simulink library "Suspension_Utilities"  (R2025a)
settings: Solver=VariableStepAuto  StartTime=0.0  StopTime=10.0  RelTol=1e-3
undefined symbols (not defined in the file or in its folder): Ac, Af, Ar, hp1, hp2, hp3, hp_in, hp_in_f_ua, hp_in_r_ua, hp_mount_subframe, hp_shk_frame, hp_spr_bot, hp_spr_top, hpb, hpf, hpo, hpx, hpz, Newton, Raphson, rotYAxis, SubframeConnection, Upper_Arm_to_Subframe, Visual, X, Y, Z
libraries: sm_lib x75, $bdroot x23, linkage_bushing_6DOF_lib x13, fl_lib x4, sharedtransformsys x3, linkage_bushing_5DOF_lib x2, nesl_utility x1
(part 1 of 3)
Description:
  | Simscape Vehicle Templates Library
  | 
  | Copyright 2018-2026 The MathWorks, Inc.
settings Model: Creator=smiller  LastModifiedBy=smiller
settings OptimizationCC: ReuseModelBlockBuffer=off
settings ModelReferenceCC: EnableRefExpFcnMdlSchedulingChecks=on
settings RTWCC: GPUComputeCapability=3.5

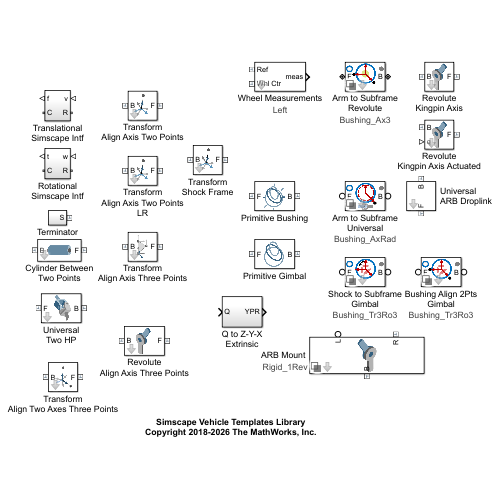
[thumbnail: Simulink's stored preview of the top-level diagram]
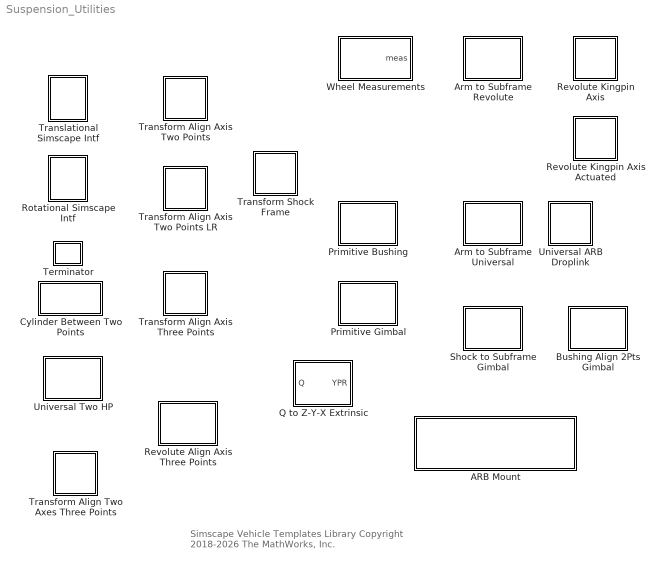
== system Suspension_Utilities ==
  note: Simscape Vehicle Templates Library
      | Copyright 2018-2026 The MathWorks, Inc.
  ARB Mount : Subsystem  Variant=on  VariantControlMode=label  VariantControl=Choice  LabelModeActiveChoice=Rigid_1Rev  mask{Connection=SubframeConnection, VariantLabel=SubframeConnection.class.Value}
      mask prompts: Connection "Connection Parameters"; VariantLabel "Variant Label"
      mask init:
      | curblk = gcb;
      | 
      | % Set variant for this block 
      | set_param(curblk,'LabelModeActiveChoice',VariantLabel);
      settings: AttributesFormatString=%<LabelModeActiveChoice>
  Arm to Subframe Revolute : Subsystem  Variant=on  VariantControlMode=label  VariantControl=Variant1  LabelModeActiveChoice=Bushing_Ax3  mask{popup_leftRight=Left, hp_f=hp_in_f_ua, hp_r=hp_in_r_ua, Connection=Upper_Arm_to_Subframe, VariantLabel=Upper_Arm_to_Subframe.class.Value}
      mask prompts: popup_leftRight "Left/Right"; hp_f "HP Front [x y z] (m)"; hp_r "HP Rear [x y z] (m)"; Connection "Connection Parameters"; VariantLabel "Variant Label"
      mask init:
      | curblk = gcb;
      | 
      | % Set variant for this block 
      | set_param(curblk,'LabelModeActiveChoice',VariantLabel);
      | 
      | if(popup_leftRight == 1)
      |     rhs_y = 1;
      | elseif(popup_leftRight == 2)
      |     rhs_y = -1;
      | end
      | 
      | rhs_hp = [1 rhs_y 1];
      settings: AttributesFormatString=%<ActiveVariant>
      mask TypeOptions popup_leftRight: Left | Right
      mask Display:
      | curblk = gcb;
      | activeVar = get_param(curblk,'activevariant');
      | ActiveVarCmd = get_param([curblk '/' strrep(activeVar,'_',' ')],'MaskDisplay');
      | eval(ActiveVarCmd);
  Arm to Subframe Universal : Subsystem  Variant=on  VariantControlMode=label  VariantControl=Variant1  LabelModeActiveChoice=Bushing_AxRad  mask(Universal Joint (Kinematic) or Compliant Element){popup_leftRight=Left, hp_joint=hp_in_f_ua, Connection=Upper_Arm_to_Subframe, VariantLabel=Upper_Arm_to_Subframe.class.Value, checkbox_setTargets=off}
      mask prompts: popup_leftRight "Left/Right"; hp_joint "Joint HP [x  y z] (m)"; Connection "Connection Parameters"; VariantLabel "Variant Label"; checkbox_setTargets "Set position targets to 0"
      mask help: Configurable part connection permitting two rotational degrees of freedom (Universal Joint) or a compliant connection. If "Right" is selected, y components will have their sign flipped.
      mask init:
      | curblk = gcb;
      | 
      | % Set variant for this block 
      | set_param(curblk,'LabelModeActiveChoice',VariantLabel);
      | 
      | set_param([curblk '/' strrep(VariantLabel,'_',' ')],'checkbox_setTargets',checkbox_setTargets);
      | 
      | if(popup_leftRight == 1)
      |     rhs_y = 1;
      | elseif(popup_leftRight == 2)
      |     rhs_y = -1;
      | end
      | 
      | rhs_hp = [1 rhs_y 1];
      settings: AttributesFormatString=%<ActiveVariant>
      mask TypeOptions popup_leftRight: Left | Right
  Bushing Align 2Pts Gimbal : Subsystem  Variant=on  VariantControlMode=label  VariantControl=Variant1  LabelModeActiveChoice=Bushing_Tr3Ro3  mask(Gimbal Joint (Kinematic) or Compliant Element){popup_leftRight=Left, hp_joint=0, Connection=Upper_Arm_to_Subframe, VariantLabel=Upper_Arm_to_Subframe.class.Value, checkbox_setTargets=off}
      mask prompts: popup_leftRight "Left/Right"; hp_joint "Joint HP [xyz] (m)"; Connection "Connection Parameters"; VariantLabel "Variant Label"; checkbox_setTargets "Set bushing joint targets to 0"
      mask help: Configurable part connection permitting three rotational degrees of freedom (Gimbal Joint) or a compliant connection. If "Right" is selected, y components will have their sign flipped.
      mask init:
      | curblk = gcb;
      | 
      | % Set variant for this block 
      | set_param(curblk,'LabelModeActiveChoice',VariantLabel);
      | 
      | if(popup_leftRight == 1)
      |     rhs_y = 1;
      | elseif(popup_leftRight == 2)
      |     rhs_y = -1;
      | end
      | 
      | rhs_hp = [1 rhs_y 1];
      | 
      | set_param([curblk '/Bushing Tr3Ro3'],'checkbox_setTargets',checkbox_setTargets);
      settings: AttributesFormatString=%<ActiveVariant>
      mask TypeOptions popup_leftRight: Left | Right
      mask Display:
      | curblk = gcb;
      | activeVar = get_param(curblk,'activevariant');
      | ActiveVarCmd = get_param([curblk '/' strrep(activeVar,'_',' ')],'MaskDisplay');
      | eval(ActiveVarCmd);
  Cylinder Between Two Points : Subsystem  mask(Cylinder between two points){hp_b=hpb, hp_f=hpf, Mass=1, clr_solid=[0.2 0.4 0.6], opc_solid=0.5, rad_solid=0.1}
      mask prompts: hp_b "Hardpoint at B [xyz] (m)"; hp_f "Hardpoint at F [xyz] (m)"; Mass "Mass (kg)"; clr_solid "Color [RGB]"; opc_solid "Opacity (0-1)"; rad_solid "Radius (m)"
      mask help: Models a cylinder parameterized by its end points.
      mask init:
      | [xftheta, xfaxis] = alignZAxisToLine(hp_b, hp_f);
      mask TypeOptions Mass: Solid/Mass
      mask TypeOptions clr_solid: Solid/GraphicDiffuseColor
      mask TypeOptions opc_solid: Solid/GraphicOpacity
      mask TypeOptions rad_solid: Solid/CylinderRadius
      mask DialogControl cont_vis Prompt: Visualization
      mask Display: image('sm_car_cylinder_two_points.png')
  Primitive Bushing : Subsystem
      mask Display: image('sm_car_primitive_bushing.png');
  Primitive Gimbal : Subsystem
      mask Display: image('sm_car_primitive_gimbal.png')
  Q to Z-Y-X Extrinsic : Subsystem
  Revolute Align Axis Three Points : Subsystem  mask(Revolute Joint 3 Points){popup_leftRight=Left, hp_1=[0 0 0], hp_2=[1 0 1], hp_3=[0 1 1], positionTargetSpecify=off, PositionTargetValue=0}
      mask prompts: popup_leftRight "Left/Right"; hp_1 "Hardpoint 1 [xyz] (m)"; hp_2 "Hardpoint 2 [xyz] (m)"; hp_3 "Hardpoint 3 [xyz] (m)"; positionTargetSpecify "Position Target Specify"; PositionTargetValue "Joint Target Value (deg)"
      mask help:
      | Revolute Joint with degree of freedom normal to 3 hardpoints.
      |
      | Positive z-axis will point along cross (HP1 -> HP3, HP1->HP2).
      mask init:
      | % Set parameter for mirroring (+y or -y)
      | if(popup_leftRight == 1)
      |     rhs_susp = 1;
      | elseif(popup_leftRight == 2)
      |     rhs_susp = -1;
      | end
      | rhs_hp = [1 rhs_susp 1];
      | 
      | if(popup_leftRight == 1)
      |     set_param([gcb '/Transform Align Axis B'],'popup_f_axis','+Z');
      |     set_param([gcb '/Transform Align Axis F'],'popup_f_axis','+Z');
      | elseif(popup_leftRight == 2)
      |     set_param([gcb '/Transform Align Axis B'],'popup_f_axis','-Z');
      |     set_param([gcb '/Transform Align Axis F'],'popup_f_axis','-Z');
      | end
      | 
      | if(get_param(gcb,'positionTargetSpecify'))
      |     set_param([gcb '/Revolute Bellcrank Pivot'],'PositionTargetSpecify','on')
      | else
      |     set_param([gcb '/Revolute Joint'],'PositionTargetSpecify','off')
      | end
      mask TypeOptions popup_leftRight: Left | Right
      mask TypeOptions PositionTargetValue:
      | Revolute
      | Bellcrank Pivot/PositionTargetValue
      mask Display: image('sm_car_variant_revolute.png')
  Revolute Kingpin Axis : Subsystem  mask{popup_leftRight=Left, aCaster=0, aKPI=0}
      mask prompts: popup_leftRight "Left/Right"; aCaster "Caster Angle (deg)"; aKPI "King Pin Inclination (KPI) Angle (deg)"
      mask init:
      | if(popup_leftRight == 1)
      |     rhs_KPIsign = 1;
      | elseif(popup_leftRight == 2)
      |     rhs_KPIsign = -1;
      | end
      mask TypeOptions popup_leftRight: Left | Right
      mask DialogControl text_caster Prompt: Positive Caster: Top Rear of WC
      mask DialogControl text_kpi Prompt: Positive KPI: Top Inside Bottom
      mask Display: image('sm_car_rev_joint_IMAGE.png');
  Revolute Kingpin Axis Actuated : Subsystem  mask{popup_leftRight=Left, aCaster=0, aKPI=0}
      mask prompts: popup_leftRight "Left/Right"; aCaster "Caster Angle (deg)"; aKPI "King Pin Inclination (KPI) Angle (deg)"
      mask init:
      | if(popup_leftRight == 1)
      |     rhs_KPIsign = 1;
      | elseif(popup_leftRight == 2)
      |     rhs_KPIsign = -1;
      | end
      mask TypeOptions popup_leftRight: Left | Right
      mask DialogControl text_caster Prompt: Positive Caster: Top Rear of WC
      mask DialogControl text_kpi Prompt: Positive KPI: Top Inside Bottom
      mask Display: image('sm_car_rev_joint_IMAGE.png');
  Rotational Simscape Intf : Subsystem
  Shock to Subframe Gimbal : Subsystem  Variant=on  VariantControlMode=label  VariantControl=Variant1  LabelModeActiveChoice=Bushing_Tr3Ro3  mask{popup_leftRight=Left, Connection=Upper_Arm_to_Subframe, VariantLabel=Upper_Arm_to_Subframe.class.Value, checkbox_setTargets=on}
      mask prompts: popup_leftRight "Left/Right"; Connection "Connection Parameters"; VariantLabel "Variant Label"; checkbox_setTargets "Set bushing joint targets to 0"
      mask init:
      | curblk = gcb;
      | 
      | % Set variant for this block 
      | set_param(curblk,'LabelModeActiveChoice',VariantLabel);
      | 
      | if(popup_leftRight == 1)
      |     rhs_y = 1;
      | elseif(popup_leftRight == 2)
      |     rhs_y = -1;
      | end
      | 
      | set_param([curblk '/Bushing Tr3Ro3'],'checkbox_setTargets',checkbox_setTargets);
      settings: AttributesFormatString=%<ActiveVariant>
      mask TypeOptions popup_leftRight: Left | Right
      mask Display:
      | curblk = gcb;
      | activeVar = get_param(curblk,'activevariant');
      | ActiveVarCmd = get_param([curblk '/' strrep(activeVar,'_',' ')],'MaskDisplay');
      | eval(ActiveVarCmd);
  Terminator : Subsystem
  Transform Align Axis Three Points : Subsystem  mask(Transform Align Axis Three Points){pt1=hp1, pt2=hp2, pt3=hp3, popup_f_axis=+Z}
      mask prompts: pt1 "Point 1 [xyz] (m)"; pt2 "Point 2 [xyz] (m)"; pt3 "Point 3 [xyz] (m)"; popup_f_axis "Axis of F Frame to Aim at Target"
      mask help: Transforms a frame to aim a selected axis along a normal to a plane defined by 3 points. All points must be defined relative to the same reference frame. Normal to the plane is defined as cross (HP1 -> HP3, HP1->HP2).
      mask init:
      | switch popup_f_axis
      |     case 1, vec = [ 1  0  0];
      |     case 2, vec = [ 0  1  0];
      |     case 3, vec = [ 0  0  1];
      |     case 4, vec = [-1  0  0];
      |     case 5, vec = [ 0 -1  0];
      |     case 6, vec = [ 0  0 -1];
      | end
      | 
      | % Unit vectors 
      | uvec1 = (pt3-pt1)/norm(pt3-pt1);
      | uvec2 = (pt2-pt1)/norm(pt2-pt1);
      | 
      | nvec = cross(uvec1,uvec2);
      | unvec = nvec/norm(nvec);
      | 
      | % Force nvec to point along +z
      | %if(unvec(3)<0)
      | %    unvec = -unvec;
      | %end
      | rotaxis = cross(vec,unvec);
      | 
      | if (norm(rotaxis)==0)
      |     if (sum(uvec1==0)==3 || sum(uvec2==0)==3)  % hps collocated
      |         rotangle = 0; 
      |     elseif ((sum(uvec1+uvec2)==0) ...  % vectors antiparallel    
      |             || (sum(vec+unvec))==0)    % vec and unvec antiparallel
      |         rotangle = pi;
      |         rotaxis = circshift(vec,1);
      |     else                       % vectors parallel
      |         rotangle = 0;          
      |     end
      | else
      |     rotangle = acos(dot(vec,unvec));
      |     %rotangle = acos(dot(vec,(hp_t-hp_b)/norm((hp_t-hp_b))))
      | end
      mask TypeOptions popup_f_axis: +X | +Y | +Z | -X | -Y | -Z
      mask Display: image('sm_car_transform_align_axis_three_points.png')
  Transform Align Axis Two Points : Subsystem  mask(Transform Align Axis Two Points){hp_b=hp1, hp_t=hp2, popup_f_axis=-Z}
      mask prompts: hp_b "Location of B [xyz] (m)"; hp_t "Target for Frame Axis [xyz] (m)"; popup_f_axis "Axis of F Frame to Aim at Target"
      mask help: Transforms a frame to aim a selected axis at a target point. Both points must be defined relative to the same reference frame.
      mask init:
      | switch popup_f_axis
      |     case 1, vec = [ 1  0  0];
      |     case 2, vec = [ 0  1  0];
      |     case 3, vec = [ 0  0  1];
      |     case 4, vec = [-1  0  0];
      |     case 5, vec = [ 0 -1  0];
      |     case 6, vec = [ 0  0 -1];
      | end
      | 
      | uvec_bt = (hp_t-hp_b)/norm(hp_t-hp_b);
      | rotaxis = cross(vec,uvec_bt);
      | 
      | if (norm(rotaxis)==0)
      |     if (uvec_bt==0)            % hps collocated
      |         rotangle = 0; 
      |     elseif ((uvec_bt+vec)==0)  % vectors antiparallel    
      |         rotangle = pi;
      |         rotaxis = circshift(vec,1);
      |     else                       % vectors parallel
      |         rotangle = 0;          
      |     end
      | else
      |     rotangle = acos(dot(vec,uvec_bt));
      |     %rotangle = acos(dot(vec,(hp_t-hp_b)/norm((hp_t-hp_b))))
      | end
      mask TypeOptions popup_f_axis: +X | +Y | +Z | -X | -Y | -Z
      mask Display: image('sm_car_transform_align_axis_two_points.png')
  Transform Align Axis Two Points LR : Subsystem  mask{popup_leftRight=Left, hp_spr_top=hp_spr_top, hp_spr_bot=hp_spr_bot}
      mask prompts: popup_leftRight "Left/Right"; hp_spr_top "Spring Top [xyz] (m)"; hp_spr_bot "Spring Bottom [xyz] (m)"
      mask init:
      | if(popup_leftRight == 1)
      |     rhs_y = 1;
      | elseif(popup_leftRight == 2)
      |     rhs_y = -1;
      | end
      | 
      | rhs_hp = [1 rhs_y 1];
      mask TypeOptions popup_leftRight: Left | Right
      mask Display: image('sm_car_transform_align_axis_two_points.png')
  Transform Align Two Axes Three Points : Subsystem  mask(Transform Align Two Axes Three Points){hpo=hpo, hpz=hpz, hpx=hpx}
      mask prompts: hpo "Origin [x y z] (m)"; hpz "Point to align z-axis [x y z] (m)"; hpx "Point to align x-axis [x y z] (m)"
      mask help: Transforms a frame to aim two selected axes to point at two provided points. All points must be defined relative to the same reference frame.
      mask init:
      | R = frameRotationFromTwoPoints(hpo, hpz, hpx);
      mask Display: image('sm_car_transform_align_two_axes_three_points.png')
  Transform Shock Frame : Subsystem  mask{popup_leftRight=Left, hp_spr_top=hp_spr_top, hp_spr_bot=hp_spr_bot, hp_shk_frame=hp_shk_frame}
      mask prompts: popup_leftRight "Left/Right"; hp_spr_top "Shock Top [xyz] (m)"; hp_spr_bot "Shock Bottom [xyz] (m)"; hp_shk_frame "Shock Frame [xyz] (m)"
      mask init:
      | if(popup_leftRight == 1)
      |     rhs_y = 1;
      | elseif(popup_leftRight == 2)
      |     rhs_y = -1;
      | end
      | 
      | vecBotTop = hp_spr_top-hp_spr_bot;
      | 
      | qx = atan2(vecBotTop(2),vecBotTop(3));
      | qy = atan2(vecBotTop(1),vecBotTop(3));
      | 
      | R = frameRotationXYextr(qx*rhs_y,qy);
      mask TypeOptions popup_leftRight: Left | Right
      mask Display: image('sm_car_transform_align_axis_two_points.png')
  Translational Simscape Intf : Subsystem
  Universal ARB Droplink : Subsystem  mask{rotYAxis=rotYAxis}
      mask prompts: rotYAxis "Universal Y Rotation (deg)"
  Universal Two HP : Subsystem  mask{popup_leftRight=Left, hp_f=hp_in_f_ua, hp_r=hp_in_r_ua}
      mask prompts: popup_leftRight "Left/Right"; hp_f "HP Front [xyz] (m)"; hp_r "HP Rear [xyz] (m)"
      mask init:
      | if(popup_leftRight == 1)
      |     rhs_y = 1;
      | elseif(popup_leftRight == 2)
      |     rhs_y = -1;
      | end
      | 
      | rhs_hp = [1 rhs_y 1];
      mask TypeOptions popup_leftRight: Left | Right
      mask Display: image('sm_car_variant_universal.png');
  Wheel Measurements : Subsystem  mask(Wheel Measurements){popup_leftRight=Left}
      mask prompts: popup_leftRight "Left/Right"
      mask help: Calculates toe and camber angles based on orientation of wheel spin axis. To estimate steering axis inclination, the same measurements are done along the longitudinal axis (X) of the tire. Set Left/Right so that the sign of the logged toe and camber angles is associated with towards/away from vehicle center.
      mask init:
      | if(popup_leftRight == 1)
      |     rhs_tc = 1;
      | elseif(popup_leftRight == 2)
      |     rhs_tc = -1;
      | end
      settings: AttributesFormatString=%<popup_leftRight>
      mask TypeOptions popup_leftRight: Left | Right

== system Suspension_Utilities/ARB Mount ==
  Bushing Ax3 : Subsystem  VariantControl=Bushing_Ax3  mask{hp_j=hp_mount_subframe, Bushing=Connection}
      mask prompts: hp_j "Joint HP [x  y z] (m)"; Bushing "Parameters (struct)"
      mask init:
      | %{
      | set_param([gcb '/Bushing L'],...
      |     'popup_force_law_spr_axiX', sprx.Law.Value,...
      |     'popup_force_law_spr_axiY', spry.Law.Value,...
      |     'popup_force_law_spr_axiZ', sprz.Law.Value,...
      |     'popup_force_law_dam_axiX', damx.Law.Value,...
      |     'popup_force_law_dam_axiY', damy.Law.Value,...
      |     'popup_force_law_dam_axiZ', damz.Law.Value...
      |     );
      | 
      | set_param([gcb '/Bushing R'],...
      |     'popup_force_law_spr_axiX', sprx.Law.Value,...
      |     'popup_force_law_spr_axiY', spry.Law.Value,...
      |     'popup_force_law_spr_axiZ', sprz.Law.Value,...
      |     'popup_force_law_dam_axiX', damx.Law.Value,...
      |     'popup_force_law_dam_axiY', damy.Law.Value,...
      |     'popup_force_law_dam_axiZ', damz.Law.Value...
      |     );
      | %}
      mask Display: image('sm_car_subframe_arb_bushing_2tra_perpaxial.png');
  Bushing Tr3Ro3 : Subsystem  VariantControl=Bushing_Tr3Ro3  mask{Bushing=Connection, sprx_law=Connection.SpringX.Law.Value, spry_law=Connection.SpringY.Law.Value, sprz_law=Connection.SpringZ.Law.Value, damx_law=Connection.DamperX.Law.Value, damy_law=Connection.DamperY.Law.Value, damz_law=Connection.DamperZ.Law.Value, sprx_law_rot=Connection.SpringX.Law.Value, spry_law_rot=Connection.SpringY.Law.Value, sprz_law_rot=Connection.SpringZ.Law.Value, damx_law_rot=Connection.DamperX.Law.Value, damy_law_rot=Connection.DamperY.Law.Value, damz_law_rot=Connection.DamperZ.Law.Value}
      mask prompts: Bushing "Parameters (struct)"; sprx_law "Spring X Force Law"; spry_law "Spring Y Force Law"; sprz_law "Spring Z Force Law"; damx_law "Damper X Force Law"; damy_law "Damper Y Force Law"; damz_law "Damper Z Force Law"; sprx_law_rot "Spring X Force Law"; spry_law_rot "Spring Y Force Law"; sprz_law_rot "Spring Z Force Law"; damx_law_rot "Damper X Force Law"; damy_law_rot "Damper Y Force Law"; damz_law_rot "Damper Z Force Law"
      mask init:
      | %{
      | set_param([gcb '/Bushing L'],...
      |     'popup_force_law_spr_axiX', sprx_law,...
      |     'popup_force_law_spr_axiY', spry_law,...
      |     'popup_force_law_spr_axiZ', sprz_law,...
      |     'popup_force_law_dam_axiX', damx_law,...
      |     'popup_force_law_dam_axiY', damy_law,...
      |     'popup_force_law_dam_axiZ', damz_law,...
      |     'popup_force_law_spr_torX', sprx_law_rot,...
      |     'popup_force_law_spr_torY', spry_law_rot,...
      |     'popup_force_law_spr_torZ', sprz_law_rot,...
      |     'popup_force_law_dam_torX', damx_law_rot,...
      |     'popup_force_law_dam_torY', damy_law_rot,...
      |     'popup_force_law_dam_torZ', damz_law_rot...
      |     );
      | 
      | set_param([gcb '/Bushing R'],...
      |     'popup_force_law_spr_axiX', sprx_law,...
      |     'popup_force_law_spr_axiY', spry_law,...
      |     'popup_force_law_spr_axiZ', sprz_law,...
      |     'popup_force_law_dam_axiX', damx_law,...
      |     'popup_force_law_dam_axiY', damy_law,...
      |     'popup_force_law_dam_axiZ', damz_law,...
      |     'popup_force_law_spr_torX', sprx_law_rot,...
      |     'popup_force_law_spr_torY', spry_law_rot,...
      |     'popup_force_law_spr_torZ', sprz_law_rot,...
      |     'popup_force_law_dam_torX', damx_law_rot,...
      |     'popup_force_law_dam_torY', damy_law_rot,...
      |     'popup_force_law_dam_torZ', damz_law_rot...
      |     );
      | %}
      mask DialogControl cont_trans Prompt: Translational
      mask DialogControl cont_rot Prompt: Rotational
      mask Display: image('sm_car_subframe_arb_bushing_2tra3rot_qz.png');
  Rigid 1Rev : Subsystem  VariantControl=Rigid_1Rev
      mask Display: image('sm_car_subframe_arb_rev.png');
  L : PMIOPort  Side=Right
  R : PMIOPort  Port=2  Side=Right
  B : PMIOPort  Port=3  Side=Left

== system Suspension_Utilities/Arm to Subframe Revolute ==
  Bushing Ax3 : Subsystem  VariantControl=Bushing_Ax3  mask{Bushing=Connection}
      mask prompts: Bushing "Parameters (struct)"
      mask Display: image('sm_car_bushing_tr3_perpaxial.png');
  Bushing AxRad : Subsystem  VariantControl=Bushing_AxRad  mask{Bushing=Connection}
      mask prompts: Bushing "Parameters (struct)"
      mask Display: image('sm_car_bushing_axrad_6dof.png');
  Bushing Tr3Ro3 : Subsystem  VariantControl=Bushing_Tr3Ro3  mask{Bushing=Connection}
      mask prompts: Bushing "Parameters (struct)"
      mask Display: image('sm_car_bushing_tr3ro3_2pts.png');
  Rigid 1Rev : Subsystem  VariantControl=Rigid_1Rev
      mask Display: image('sm_car_variant_revolute.png')
  Rigid 2Rev : Subsystem  VariantControl=Rigid_2Rev
      mask Display: image('sm_car_variant_revolute_2rev.png');
  F : PMIOPort  Side=Right
  " B" : PMIOPort  Port=2  Side=Left

== system Suspension_Utilities/Arm to Subframe Universal ==
  Bushing Ax3 : linkage_bushing_5DOF_lib/Bushing Ax3  VariantControl=Bushing_Ax3  leftOrRight=rhs_y  hp_j=hp_joint  checkbox_setTargets=on  hp_z=Connection.sAxialOrientationZ.Value  hp_x=Connection.sAxialOrientationX.Value  AxisAttachment=Connection.AxisAttachment.class.Value  sprx=Connection.SpringX  spry=Connection.SpringY  sprz=Connection.SpringZ  damx=Connection.DamperX  damy=Connection.DamperY  damz=Connection.DamperZ  shell_or=Visual.hp.rad*2  shell_ir=Visual.hp.rad  shell_len=Visual.hp.rad*2  elastomer_clr=Visual.Bushing.clr  elastomer_opc=Visual.part.opc  shell_clr=Visual.BushingShell.clr  shell_opc=Visual.part.opc  sleeve_clr=Visual.Bushing.clr  sleeve_opc=Visual.part.opc
  Bushing AxRad : linkage_bushing_5DOF_lib/Bushing AxRad  VariantControl=Bushing_AxRad  leftOrRight=rhs_y  hp_j=hp_joint  checkbox_setTargets=on  hp_z=Connection.sAxialOrientation.Value  sprRad=Connection.RadialSpring  damRad=Connection.RadialDamper  sprAxi=Connection.AxialSpring  damAxi=Connection.AxialDamper  shell_or=Visual.hp.rad*2  shell_len=Visual.hp.rad*2  shell_clr=Visual.BushingShell.clr  shell_opc=Visual.part.opc  sleeve_clr=Visual.Bushing.clr  sleeve_opc=Visual.part.opc
  Bushing Tr3Ro3 : linkage_bushing_6DOF_lib/Bushing Tr3Ro3 2Pts  VariantControl=Bushing_Tr3Ro3  checkbox_setTargets=off  leftOrRight=rhs_y  hp_j=hp_joint  hp_z=Connection.sAxialOrientationZ.Value  hp_x=Connection.sAxialOrientationX.Value  sprx=Connection.SpringX  spry=Connection.SpringY  sprz=Connection.SpringZ  damx=Connection.DamperX  damy=Connection.DamperY  damz=Connection.DamperZ  sprqx=Connection.SpringqX  sprqy=Connection.SpringqY  sprqz=Connection.SpringqZ  damqx=Connection.DamperqX  damqy=Connection.DamperqY  damqz=Connection.DamperqZ  shell_or=Visual.hp.rad*2  shell_len=Visual.hp.rad*2  shell_clr=Visual.BushingShell.clr  shell_opc=Visual.part.opc  sleeve_clr=Visual.Bushing.clr  sleeve_opc=Visual.part.opc
  Rigid UJ : Subsystem  VariantControl=Rigid_UJ  mask{popup_leftRight=Left, checkbox_setTargets=on}
      mask prompts: popup_leftRight "Left/Right"; checkbox_setTargets "Set position targets to 0"
      mask init:
      | curblk = gcb;
      | 
      | if(popup_leftRight == 1)
      |     rhs_y = 1;
      | elseif(popup_leftRight == 2)
      |     rhs_y = -1;
      | end
      | 
      | rhs_hp = [1 rhs_y 1];
      | 
      | if(checkbox_setTargets)
      |     set_param([curblk '/Universal Joint'],...
      |         'RxPositionTargetSpecify','on',...
      |         'RyPositionTargetSpecify','on'...
      |         );
      | else
      |     set_param([curblk '/Universal Joint'],...
      |         'RxPositionTargetSpecify','off',...
      |         'RyPositionTargetSpecify','off'...
      |         );
      | end
      mask TypeOptions popup_leftRight: Left | Right
      mask Display: image('sm_car_variant_universal.png');
  F : PMIOPort  Side=Right
  " B" : PMIOPort  Port=2  Side=Left

== system Suspension_Utilities/Bushing Align 2Pts Gimbal ==
  Bushing Tr3Ro3 : linkage_bushing_6DOF_lib/Bushing Tr3Ro3 2Pts  VariantControl=Bushing_Tr3Ro3  checkbox_setTargets=on  leftOrRight=rhs_y  hp_j=hp_joint  hp_z=Connection.sAxialOrientationZ.Value  hp_x=Connection.sAxialOrientationX.Value  sprx=Connection.SpringX  spry=Connection.SpringY  sprz=Connection.SpringZ  damx=Connection.DamperX  damy=Connection.DamperY  damz=Connection.DamperZ  sprqx=Connection.SpringqX  sprqy=Connection.SpringqY  sprqz=Connection.SpringqZ  damqx=Connection.DamperqX  damqy=Connection.DamperqY  damqz=Connection.DamperqZ  shell_or=Visual.hp.rad*2  shell_len=Visual.hp.rad*2  shell_clr=Visual.BushingShell.clr  shell_opc=Visual.part.opc  sleeve_clr=Visual.Bushing.clr  sleeve_opc=Visual.part.opc
  Rigid Gimbal : Subsystem  VariantControl=Rigid_Gimbal
      mask Display: image('sm_car_variant_bushing_gimbal.png')
  F : PMIOPort  Side=Right
  " B" : PMIOPort  Port=2  Side=Left

== system Suspension_Utilities/Cylinder Between Two Points ==
  Solid : sm_lib/Body Elements/Cylindrical Solid  CylinderRadius=rad_solid  CylinderRadiusUnits=m  CylinderLength=norm(hp_f-hp_b)  CylinderLengthUnits=m  ExportEntireGeometry=off  InertiaType=CalculateFromGeometry  BasedOnType=Mass  Density=1000  DensityUnits=kg/m^3  Mass=Mass  MassUnits=kg  CenterOfMass=[0 0 0]  CenterOfMassUnits=m  MomentsOfInertia=[1 1 1]  MomentsOfInertiaUnits=kg*m^2  ProductsOfInertia=[0 0 0]  ProductsOfInertiaUnits=kg*m^2  GraphicType=FromGeometry  MarkerShape=Sphere  MarkerSize=10  GraphicVisPropType=SimpleVisualProperties  GraphicDiffuseColor=clr_solid  GraphicOpacity=opc_solid  GraphicSpecularColor=[0.5 0.5 0.5 1.0]  GraphicAmbientColor=[0.15 0.15 0.15 1.0]  GraphicEmissiveColor=[0.0 0.0 0.0 1.0]  GraphicShininess=75  DoExposeReferenceFrame=on  SerializedFrames=<Frames/>
  Transform Align Z B to F : sm_lib/Frames and Transforms/Rigid Transform  RotationMethod=ArbitraryAxis  FollAlignAxisA=+X  BaseAlignAxisA=+Y  FollAlignAxisB=+Y  BaseAlignAxisB=+Z  RotationStandardAxis=+Z  RotationAngle=xftheta  RotationAngleUnits=rad  RotationArbitraryAxis=xfaxis  RotationSequenceAxes=FollowerAxes  RotationSequence=XYX  RotationSequenceAngles=[0 0 0]  RotationSequenceAnglesUnits=deg  RotationMatrix=[1 0 0; 0 1 0; 0 0 1]  Quaternion=[1 0 0 0]  TranslationMethod=None  TranslationCartesianOffset=[0 0 0]  TranslationCartesianOffsetUnits=m  TranslationStandardAxis=+Z  TranslationStandardOffset=0  TranslationStandardOffsetUnits=m  TranslationROffset=0  TranslationROffsetUnits=m  TranslationThetaOffset=0  TranslationThetaOffsetUnits=deg  TranslationZOffset=0  TranslationZOffsetUnits=m
  Transform B to Ctr : sm_lib/Frames and Transforms/Rigid Transform  RotationMethod=None  FollAlignAxisA=+X  BaseAlignAxisA=+Y  FollAlignAxisB=+Y  BaseAlignAxisB=+Z  RotationStandardAxis=+Z  RotationAngle=0.0  RotationAngleUnits=deg  RotationArbitraryAxis=[0 0 1]  RotationSequenceAxes=FollowerAxes  RotationSequence=XYX  RotationSequenceAngles=[0 0 0]  RotationSequenceAnglesUnits=deg  RotationMatrix=[1 0 0; 0 1 0; 0 0 1]  Quaternion=[1 0 0 0]  TranslationMethod=Cartesian  TranslationCartesianOffset=0.5*(hp_f-hp_b)  TranslationCartesianOffsetUnits=m  TranslationStandardAxis=+Z  TranslationStandardOffset=0  TranslationStandardOffsetUnits=m  TranslationROffset=0  TranslationROffsetUnits=m  TranslationThetaOffset=0  TranslationThetaOffsetUnits=deg  TranslationZOffset=0  TranslationZOffsetUnits=m
  Transform Ctr to F : sm_lib/Frames and Transforms/Rigid Transform  RotationMethod=None  FollAlignAxisA=+X  BaseAlignAxisA=+Y  FollAlignAxisB=+Y  BaseAlignAxisB=+Z  RotationStandardAxis=+Z  RotationAngle=0.0  RotationAngleUnits=deg  RotationArbitraryAxis=[0 0 1]  RotationSequenceAxes=FollowerAxes  RotationSequence=XYX  RotationSequenceAngles=[0 0 0]  RotationSequenceAnglesUnits=deg  RotationMatrix=[1 0 0; 0 1 0; 0 0 1]  Quaternion=[1 0 0 0]  TranslationMethod=Cartesian  TranslationCartesianOffset=0.5*(hp_f-hp_b)  TranslationCartesianOffsetUnits=m  TranslationStandardAxis=+Z  TranslationStandardOffset=0  TranslationStandardOffsetUnits=m  TranslationROffset=0  TranslationROffsetUnits=m  TranslationThetaOffset=0  TranslationThetaOffsetUnits=deg  TranslationZOffset=0  TranslationZOffsetUnits=m
  F : PMIOPort  Side=Right
  B : PMIOPort  Port=2  Side=Left
  connections:
  Transform Ctr to F/RConn1 -- F/RConn1
  Transform Align Z B to F/RConn1 -- Solid/RConn1
  Transform Align Z B to F/LConn1 -- Transform Ctr to F/LConn1 -- Transform B to Ctr/RConn1
  Transform B to Ctr/LConn1 -- B/RConn1

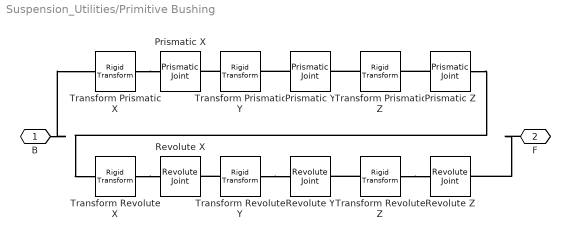
== system Suspension_Utilities/Primitive Bushing ==
  Prismatic X : sm_lib/Joints/Prismatic Joint  JointMode=Normal  CompositeWrenchDir=FollowerOnBase  CompositeWrenchFrame=BaseFrame  SenseConstraintForce=off  SenseConstraintTorque=off  SenseTotalForce=off  SenseTotalTorque=off  PositionTargetSpecify=off  PositionTargetPriority=High  PositionTargetValue=0  PositionTargetValueUnits=m  VelocityTargetSpecify=off  VelocityTargetPriority=High  VelocityTargetValue=0  VelocityTargetValueUnits=m/s  EquilibriumPosition=0  EquilibriumPositionUnits=m  SpringStiffness=0  SpringStiffnessUnits=N/m  DampingCoefficient=0  DampingCoefficientUnits=N/(m/s)  LowerLimitSpecify=off  LowerLimitBound=-1  LowerLimitBoundUnits=m  LowerLimitStiffness=1e6  LowerLimitStiffnessUnits=N/m  LowerLimitDamping=1e3  LowerLimitDampingUnits=N/(m/s)  LowerLimitTransitionRegionWidth=1e-4  LowerLimitTransitionRegionWidthUnits=m  UpperLimitSpecify=off  UpperLimitBound=1  UpperLimitBoundUnits=m  UpperLimitStiffness=1e6  UpperLimitStiffnessUnits=N/m  UpperLimitDamping=1e3  UpperLimitDampingUnits=N/(m/s)  UpperLimitTransitionRegionWidth=1e-4  UpperLimitTransitionRegionWidthUnits=m  TorqueActuationMode=NoTorque  MotionActuationMode=ComputedMotion  SensePosition=off  SenseVelocity=off  SenseAcceleration=off  SenseTorqueForce=off  SenseLowerLimitTorqueForce=off  SenseUpperLimitTorqueForce=off
  Prismatic Y : sm_lib/Joints/Prismatic Joint  JointMode=Normal  CompositeWrenchDir=FollowerOnBase  CompositeWrenchFrame=BaseFrame  SenseConstraintForce=off  SenseConstraintTorque=off  SenseTotalForce=off  SenseTotalTorque=off  PositionTargetSpecify=off  PositionTargetPriority=High  PositionTargetValue=0  PositionTargetValueUnits=m  VelocityTargetSpecify=off  VelocityTargetPriority=High  VelocityTargetValue=0  VelocityTargetValueUnits=m/s  EquilibriumPosition=0  EquilibriumPositionUnits=m  SpringStiffness=0  SpringStiffnessUnits=N/m  DampingCoefficient=0  DampingCoefficientUnits=N/(m/s)  LowerLimitSpecify=off  LowerLimitBound=-1  LowerLimitBoundUnits=m  LowerLimitStiffness=1e6  LowerLimitStiffnessUnits=N/m  LowerLimitDamping=1e3  LowerLimitDampingUnits=N/(m/s)  LowerLimitTransitionRegionWidth=1e-4  LowerLimitTransitionRegionWidthUnits=m  UpperLimitSpecify=off  UpperLimitBound=1  UpperLimitBoundUnits=m  UpperLimitStiffness=1e6  UpperLimitStiffnessUnits=N/m  UpperLimitDamping=1e3  UpperLimitDampingUnits=N/(m/s)  UpperLimitTransitionRegionWidth=1e-4  UpperLimitTransitionRegionWidthUnits=m  TorqueActuationMode=NoTorque  MotionActuationMode=ComputedMotion  SensePosition=off  SenseVelocity=off  SenseAcceleration=off  SenseTorqueForce=off  SenseLowerLimitTorqueForce=off  SenseUpperLimitTorqueForce=off
  Prismatic Z : sm_lib/Joints/Prismatic Joint  JointMode=Normal  CompositeWrenchDir=FollowerOnBase  CompositeWrenchFrame=BaseFrame  SenseConstraintForce=off  SenseConstraintTorque=off  SenseTotalForce=off  SenseTotalTorque=off  PositionTargetSpecify=off  PositionTargetPriority=High  PositionTargetValue=0  PositionTargetValueUnits=m  VelocityTargetSpecify=off  VelocityTargetPriority=High  VelocityTargetValue=0  VelocityTargetValueUnits=m/s  EquilibriumPosition=0  EquilibriumPositionUnits=m  SpringStiffness=0  SpringStiffnessUnits=N/m  DampingCoefficient=0  DampingCoefficientUnits=N/(m/s)  LowerLimitSpecify=off  LowerLimitBound=-1  LowerLimitBoundUnits=m  LowerLimitStiffness=1e6  LowerLimitStiffnessUnits=N/m  LowerLimitDamping=1e3  LowerLimitDampingUnits=N/(m/s)  LowerLimitTransitionRegionWidth=1e-4  LowerLimitTransitionRegionWidthUnits=m  UpperLimitSpecify=off  UpperLimitBound=1  UpperLimitBoundUnits=m  UpperLimitStiffness=1e6  UpperLimitStiffnessUnits=N/m  UpperLimitDamping=1e3  UpperLimitDampingUnits=N/(m/s)  UpperLimitTransitionRegionWidth=1e-4  UpperLimitTransitionRegionWidthUnits=m  TorqueActuationMode=NoTorque  MotionActuationMode=ComputedMotion  SensePosition=off  SenseVelocity=off  SenseAcceleration=off  SenseTorqueForce=off  SenseLowerLimitTorqueForce=off  SenseUpperLimitTorqueForce=off
  Revolute X : sm_lib/Joints/Revolute Joint  JointMode=Normal  CompositeWrenchDir=FollowerOnBase  CompositeWrenchFrame=BaseFrame  SenseConstraintForce=off  SenseConstraintTorque=off  SenseTotalForce=off  SenseTotalTorque=off  PositionTargetSpecify=off  PositionTargetPriority=High  PositionTargetValue=0  PositionTargetValueUnits=deg  VelocityTargetSpecify=off  VelocityTargetPriority=High  VelocityTargetValue=0  VelocityTargetValueUnits=deg/s  EquilibriumPosition=0  EquilibriumPositionUnits=deg  SpringStiffness=0  SpringStiffnessUnits=N*m/deg  DampingCoefficient=0  DampingCoefficientUnits=N*m/(deg/s)  LowerLimitSpecify=off  LowerLimitBound=-90  LowerLimitBoundUnits=deg  LowerLimitStiffness=1e4  LowerLimitStiffnessUnits=N*m/deg  LowerLimitDamping=10  LowerLimitDampingUnits=N*m/(deg/s)  LowerLimitTransitionRegionWidth=0.1  LowerLimitTransitionRegionWidthUnits=deg  UpperLimitSpecify=off  UpperLimitBound=90  UpperLimitBoundUnits=deg  UpperLimitStiffness=1e4  UpperLimitStiffnessUnits=N*m/deg  UpperLimitDamping=10  UpperLimitDampingUnits=N*m/(deg/s)  UpperLimitTransitionRegionWidth=0.1  UpperLimitTransitionRegionWidthUnits=deg  TorqueActuationMode=NoTorque  MotionActuationMode=ComputedMotion  SensePosition=off  SenseVelocity=off  SenseAcceleration=off  SenseTorqueForce=off  SenseLowerLimitTorqueForce=off  SenseUpperLimitTorqueForce=off
  Revolute Y : sm_lib/Joints/Revolute Joint  JointMode=Normal  CompositeWrenchDir=FollowerOnBase  CompositeWrenchFrame=BaseFrame  SenseConstraintForce=off  SenseConstraintTorque=off  SenseTotalForce=off  SenseTotalTorque=off  PositionTargetSpecify=off  PositionTargetPriority=High  PositionTargetValue=0  PositionTargetValueUnits=deg  VelocityTargetSpecify=off  VelocityTargetPriority=High  VelocityTargetValue=0  VelocityTargetValueUnits=deg/s  EquilibriumPosition=0  EquilibriumPositionUnits=deg  SpringStiffness=0  SpringStiffnessUnits=N*m/deg  DampingCoefficient=0  DampingCoefficientUnits=N*m/(deg/s)  LowerLimitSpecify=off  LowerLimitBound=-90  LowerLimitBoundUnits=deg  LowerLimitStiffness=1e4  LowerLimitStiffnessUnits=N*m/deg  LowerLimitDamping=10  LowerLimitDampingUnits=N*m/(deg/s)  LowerLimitTransitionRegionWidth=0.1  LowerLimitTransitionRegionWidthUnits=deg  UpperLimitSpecify=off  UpperLimitBound=90  UpperLimitBoundUnits=deg  UpperLimitStiffness=1e4  UpperLimitStiffnessUnits=N*m/deg  UpperLimitDamping=10  UpperLimitDampingUnits=N*m/(deg/s)  UpperLimitTransitionRegionWidth=0.1  UpperLimitTransitionRegionWidthUnits=deg  TorqueActuationMode=NoTorque  MotionActuationMode=ComputedMotion  SensePosition=off  SenseVelocity=off  SenseAcceleration=off  SenseTorqueForce=off  SenseLowerLimitTorqueForce=off  SenseUpperLimitTorqueForce=off
  Revolute Z : sm_lib/Joints/Revolute Joint  JointMode=Normal  CompositeWrenchDir=FollowerOnBase  CompositeWrenchFrame=BaseFrame  SenseConstraintForce=off  SenseConstraintTorque=off  SenseTotalForce=off  SenseTotalTorque=off  PositionTargetSpecify=off  PositionTargetPriority=High  PositionTargetValue=0  PositionTargetValueUnits=deg  VelocityTargetSpecify=off  VelocityTargetPriority=High  VelocityTargetValue=0  VelocityTargetValueUnits=deg/s  EquilibriumPosition=0  EquilibriumPositionUnits=deg  SpringStiffness=0  SpringStiffnessUnits=N*m/deg  DampingCoefficient=0  DampingCoefficientUnits=N*m/(deg/s)  LowerLimitSpecify=off  LowerLimitBound=-90  LowerLimitBoundUnits=deg  LowerLimitStiffness=1e4  LowerLimitStiffnessUnits=N*m/deg  LowerLimitDamping=10  LowerLimitDampingUnits=N*m/(deg/s)  LowerLimitTransitionRegionWidth=0.1  LowerLimitTransitionRegionWidthUnits=deg  UpperLimitSpecify=off  UpperLimitBound=90  UpperLimitBoundUnits=deg  UpperLimitStiffness=1e4  UpperLimitStiffnessUnits=N*m/deg  UpperLimitDamping=10  UpperLimitDampingUnits=N*m/(deg/s)  UpperLimitTransitionRegionWidth=0.1  UpperLimitTransitionRegionWidthUnits=deg  TorqueActuationMode=NoTorque  MotionActuationMode=ComputedMotion  SensePosition=off  SenseVelocity=off  SenseAcceleration=off  SenseTorqueForce=off  SenseLowerLimitTorqueForce=off  SenseUpperLimitTorqueForce=off
  Transform Prismatic X : sm_lib/Frames and Transforms/Rigid Transform  RotationMethod=AlignedAxes  FollAlignAxisA=+Z  BaseAlignAxisA=+X  FollAlignAxisB=+Y  BaseAlignAxisB=+Y  RotationStandardAxis=+Z  RotationAngle=0.0  RotationAngleUnits=deg  RotationArbitraryAxis=[0 0 1]  RotationSequenceAxes=FollowerAxes  RotationSequence=XYX  RotationSequenceAngles=[0 0 0]  RotationSequenceAnglesUnits=deg  RotationMatrix=[1 0 0; 0 1 0; 0 0 1]  Quaternion=[1 0 0 0]  TranslationMethod=None  TranslationCartesianOffset=[0 0 0]  TranslationCartesianOffsetUnits=m  TranslationStandardAxis=+Z  TranslationStandardOffset=0  TranslationStandardOffsetUnits=m  TranslationROffset=0  TranslationROffsetUnits=m  TranslationThetaOffset=0  TranslationThetaOffsetUnits=deg  TranslationZOffset=0  TranslationZOffsetUnits=m
  Transform Prismatic Y : sm_lib/Frames and Transforms/Rigid Transform  RotationMethod=AlignedAxes  FollAlignAxisA=+Z  BaseAlignAxisA=+Y  FollAlignAxisB=+X  BaseAlignAxisB=+Z  RotationStandardAxis=+Z  RotationAngle=0.0  RotationAngleUnits=deg  RotationArbitraryAxis=[0 0 1]  RotationSequenceAxes=FollowerAxes  RotationSequence=XYX  RotationSequenceAngles=[0 0 0]  RotationSequenceAnglesUnits=deg  RotationMatrix=[1 0 0; 0 1 0; 0 0 1]  Quaternion=[1 0 0 0]  TranslationMethod=None  TranslationCartesianOffset=[0 0 0]  TranslationCartesianOffsetUnits=m  TranslationStandardAxis=+Z  TranslationStandardOffset=0  TranslationStandardOffsetUnits=m  TranslationROffset=0  TranslationROffsetUnits=m  TranslationThetaOffset=0  TranslationThetaOffsetUnits=deg  TranslationZOffset=0  TranslationZOffsetUnits=m
  Transform Prismatic Z : sm_lib/Frames and Transforms/Rigid Transform  RotationMethod=AlignedAxes  FollAlignAxisA=+Y  BaseAlignAxisA=+Z  FollAlignAxisB=+X  BaseAlignAxisB=+X  RotationStandardAxis=+Z  RotationAngle=0.0  RotationAngleUnits=deg  RotationArbitraryAxis=[0 0 1]  RotationSequenceAxes=FollowerAxes  RotationSequence=XYX  RotationSequenceAngles=[0 0 0]  RotationSequenceAnglesUnits=deg  RotationMatrix=[1 0 0; 0 1 0; 0 0 1]  Quaternion=[1 0 0 0]  TranslationMethod=None  TranslationCartesianOffset=[0 0 0]  TranslationCartesianOffsetUnits=m  TranslationStandardAxis=+Z  TranslationStandardOffset=0  TranslationStandardOffsetUnits=m  TranslationROffset=0  TranslationROffsetUnits=m  TranslationThetaOffset=0  TranslationThetaOffsetUnits=deg  TranslationZOffset=0  TranslationZOffsetUnits=m
  Transform Revolute X : sm_lib/Frames and Transforms/Rigid Transform  RotationMethod=AlignedAxes  FollAlignAxisA=+Z  BaseAlignAxisA=+X  FollAlignAxisB=+Y  BaseAlignAxisB=+Y  RotationStandardAxis=+Z  RotationAngle=0.0  RotationAngleUnits=deg  RotationArbitraryAxis=[0 0 1]  RotationSequenceAxes=FollowerAxes  RotationSequence=XYX  RotationSequenceAngles=[0 0 0]  RotationSequenceAnglesUnits=deg  RotationMatrix=[1 0 0; 0 1 0; 0 0 1]  Quaternion=[1 0 0 0]  TranslationMethod=None  TranslationCartesianOffset=[0 0 0]  TranslationCartesianOffsetUnits=m  TranslationStandardAxis=+Z  TranslationStandardOffset=0  TranslationStandardOffsetUnits=m  TranslationROffset=0  TranslationROffsetUnits=m  TranslationThetaOffset=0  TranslationThetaOffsetUnits=deg  TranslationZOffset=0  TranslationZOffsetUnits=m
  Transform Revolute Y : sm_lib/Frames and Transforms/Rigid Transform  RotationMethod=AlignedAxes  FollAlignAxisA=+Z  BaseAlignAxisA=+Y  FollAlignAxisB=+X  BaseAlignAxisB=+Z  RotationStandardAxis=+Z  RotationAngle=0.0  RotationAngleUnits=deg  RotationArbitraryAxis=[0 0 1]  RotationSequenceAxes=FollowerAxes  RotationSequence=XYX  RotationSequenceAngles=[0 0 0]  RotationSequenceAnglesUnits=deg  RotationMatrix=[1 0 0; 0 1 0; 0 0 1]  Quaternion=[1 0 0 0]  TranslationMethod=None  TranslationCartesianOffset=[0 0 0]  TranslationCartesianOffsetUnits=m  TranslationStandardAxis=+Z  TranslationStandardOffset=0  TranslationStandardOffsetUnits=m  TranslationROffset=0  TranslationROffsetUnits=m  TranslationThetaOffset=0  TranslationThetaOffsetUnits=deg  TranslationZOffset=0  TranslationZOffsetUnits=m
  Transform Revolute Z : sm_lib/Frames and Transforms/Rigid Transform  RotationMethod=AlignedAxes  FollAlignAxisA=+Y  BaseAlignAxisA=+Z  FollAlignAxisB=+X  BaseAlignAxisB=+X  RotationStandardAxis=+Z  RotationAngle=0.0  RotationAngleUnits=deg  RotationArbitraryAxis=[0 0 1]  RotationSequenceAxes=FollowerAxes  RotationSequence=XYX  RotationSequenceAngles=[0 0 0]  RotationSequenceAnglesUnits=deg  RotationMatrix=[1 0 0; 0 1 0; 0 0 1]  Quaternion=[1 0 0 0]  TranslationMethod=None  TranslationCartesianOffset=[0 0 0]  TranslationCartesianOffsetUnits=m  TranslationStandardAxis=+Z  TranslationStandardOffset=0  TranslationStandardOffsetUnits=m  TranslationROffset=0  TranslationROffsetUnits=m  TranslationThetaOffset=0  TranslationThetaOffsetUnits=deg  TranslationZOffset=0  TranslationZOffsetUnits=m
  B : PMIOPort  Side=Left
  F : PMIOPort  Port=2  Side=Right
  connections:
  Transform Prismatic Z/LConn1 -- Prismatic Y/RConn1
  Transform Revolute Y/LConn1 -- Revolute X/RConn1
  F/RConn1 -- Revolute Z/RConn1
  Transform Revolute Z/LConn1 -- Revolute Y/RConn1
  Transform Revolute X/RConn1 -- Revolute X/LConn1
  Transform Revolute Y/RConn1 -- Revolute Y/LConn1
  Prismatic Y/LConn1 -- Transform Prismatic Y/RConn1
  Transform Revolute Z/RConn1 -- Revolute Z/LConn1
  Transform Prismatic Y/LConn1 -- Prismatic X/RConn1
  Prismatic Z/LConn1 -- Transform Prismatic Z/RConn1
  Prismatic Z/RConn1 -- Transform Revolute X/LConn1
  Transform Prismatic X/RConn1 -- Prismatic X/LConn1
  B/RConn1 -- Transform Prismatic X/LConn1
